simulink model "drive_system"  (R2026b)
settings: Solver=VariableStepAuto
undefined symbols (not defined in the file or in its folder): P, Ts
settings Model: Creator=aomar  LastModifiedBy=aomar

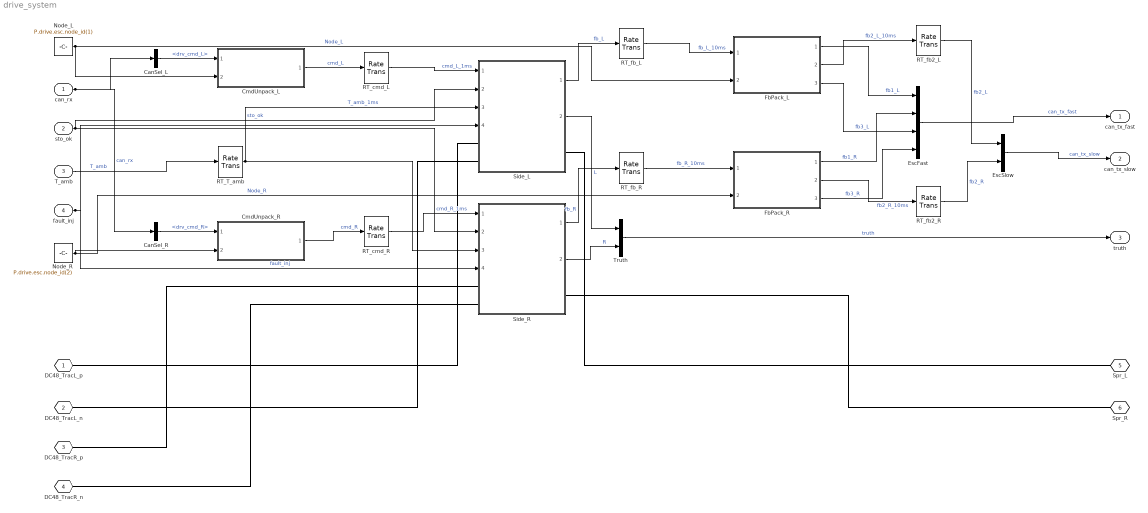
== system drive_system ==
  can_rx : Inport  OutDataTypeStr=Bus: Bus_Can1_McuFast  SampleTime=Ts.can_drive
  sto_ok : Inport  Port=2  OutDataTypeStr=boolean  SampleTime=Ts.base
  T_amb : Inport  Port=3  OutDataTypeStr=double  SampleTime=Ts.hk
  fault_inj : Inport  Port=4  OutDataTypeStr=Bus: Bus_DriveFaultInj  SampleTime=Ts.base
  CanSel_L : BusSelector  OutputSignals=drv_cmd_L
  CanSel_R : BusSelector  OutputSignals=drv_cmd_R
  CmdUnpack_L : Subsystem  ReferencedSubsystem=drive_cmd_unpack
  CmdUnpack_R : Subsystem  ReferencedSubsystem=drive_cmd_unpack
  EscFast : BusCreator  Inputs=4  OutDataTypeStr=Bus: Bus_Can1_EscFast  NonVirtualBus=on
  EscSlow : BusCreator  Inputs=2  OutDataTypeStr=Bus: Bus_Can1_EscSlow  NonVirtualBus=on
  FbPack_L : Subsystem  ReferencedSubsystem=drive_fb_pack
  FbPack_R : Subsystem  ReferencedSubsystem=drive_fb_pack
  Node_L : Constant  Value=P.drive.esc.node_id(1)  OutDataTypeStr=uint8
  Node_R : Constant  Value=P.drive.esc.node_id(2)  OutDataTypeStr=uint8
  RT_T_amb : RateTransition  InitialCondition=P.drive.thermal.T_amb0  OutPortSampleTime=Ts.base
  RT_cmd_L : RateTransition  OutPortSampleTime=Ts.esc
  RT_cmd_R : RateTransition  OutPortSampleTime=Ts.esc
  RT_fb2_L : RateTransition  OutPortSampleTime=Ts.can_fb2
  RT_fb2_R : RateTransition  OutPortSampleTime=Ts.can_fb2
  RT_fb_L : RateTransition  OutPortSampleTime=Ts.can_drive
  RT_fb_R : RateTransition  OutPortSampleTime=Ts.can_drive
  Side_L : Subsystem  ReferencedSubsystem=drive_side  side=1
  Side_R : Subsystem  ReferencedSubsystem=drive_side  side=2
  Truth : BusCreator  Inputs=2  OutDataTypeStr=Bus: Bus_DriveTruth  NonVirtualBus=on
  DC48_TracL_p : PMIOPort  Side=Left  ConnectionType=Connection: foundation.electrical.electrical
  DC48_TracL_n : PMIOPort  Port=2  Side=Left  ConnectionType=Connection: foundation.electrical.electrical
  DC48_TracR_p : PMIOPort  Port=3  Side=Left  ConnectionType=Connection: foundation.electrical.electrical
  DC48_TracR_n : PMIOPort  Port=4  Side=Left  ConnectionType=Connection: foundation.electrical.electrical
  Spr_L : PMIOPort  Port=5  Side=Right  ConnectionType=Connection: foundation.mechanical.rotational.rotational
  Spr_R : PMIOPort  Port=6  Side=Right  ConnectionType=Connection: foundation.mechanical.rotational.rotational
  can_tx_fast : Outport  OutDataTypeStr=Bus: Bus_Can1_EscFast  SampleTime=Ts.can_drive
  can_tx_slow : Outport  Port=2  OutDataTypeStr=Bus: Bus_Can1_EscSlow  SampleTime=Ts.can_fb2
  truth : Outport  Port=3  OutDataTypeStr=Bus: Bus_DriveTruth  SampleTime=Ts.base
  wires:
  Node_L/1 -> FbPack_L/2, CmdUnpack_L/2  "Node_L"
  can_rx/1 -> CanSel_R/1, CanSel_L/1  "can_rx"
  sto_ok/1 -> Side_R/2, Side_L/2  "sto_ok"
  T_amb/1 -> RT_T_amb/1  "T_amb"
  CanSel_L/1 -> CmdUnpack_L/1  "<drv_cmd_L>"
  CanSel_R/1 -> CmdUnpack_R/1  "<drv_cmd_R>"
  RT_T_amb/1 -> Side_R/3, Side_L/3  "T_amb_1ms"
  CmdUnpack_L/1 -> RT_cmd_L/1  "cmd_L"
  CmdUnpack_R/1 -> RT_cmd_R/1  "cmd_R"
  RT_cmd_L/1 -> Side_L/1  "cmd_L_1ms"
  RT_cmd_R/1 -> Side_R/1  "cmd_R_1ms"
  Side_L/1 -> RT_fb_L/1  "fb_L"
  Side_L/2 -> Truth/1  "L"
  Side_R/1 -> RT_fb_R/1  "fb_R"
  Side_R/2 -> Truth/2  "R"
  Truth/1 -> truth/1  "truth"
  RT_fb_L/1 -> FbPack_L/1  "fb_L_10ms"
  RT_fb_R/1 -> FbPack_R/1  "fb_R_10ms"
  FbPack_L/1 -> EscFast/1  "fb1_L"
  FbPack_L/2 -> RT_fb2_L/1  "fb2_L_10ms"
  FbPack_L/3 -> EscFast/3  "fb3_L"
  FbPack_R/1 -> EscFast/2  "fb1_R"
  FbPack_R/2 -> RT_fb2_R/1  "fb2_R_10ms"
  FbPack_R/3 -> EscFast/4  "fb3_R"
  EscFast/1 -> can_tx_fast/1  "can_tx_fast"
  RT_fb2_L/1 -> EscSlow/1  "fb2_L"
  RT_fb2_R/1 -> EscSlow/2  "fb2_R"
  EscSlow/1 -> can_tx_slow/1  "can_tx_slow"
  fault_inj/1 -> Side_L/4, Side_R/4  "fault_inj"
  Node_R/1 -> FbPack_R/2, CmdUnpack_R/2  "Node_R"
  connections:
  DC48_TracL_n/RConn1 -- Side_L/LConn2
  DC48_TracL_p/RConn1 -- Side_L/LConn1
  DC48_TracR_n/RConn1 -- Side_R/LConn2
  DC48_TracR_p/RConn1 -- Side_R/LConn1
  Side_L/RConn1 -- Spr_L/RConn1
  Side_R/RConn1 -- Spr_R/RConn1
